simulink model "reachout_sample_spring"  (Simulink 8.1)
settings: Solver=ode4  SolverMode=SingleTasking  StartTime=0.0  StopTime=inf  FixedStep=0.0005  RelTol=1e-3
model workspace (MAT data in the model file):
  BKIN_STEP_TIME = 0.0005
  col_x = 1
  col_y = 2
  E_STAY_CENTER = 2
  E_TARGET_ON = 3
  E_HOLD_AT_TARGET = 5
  VRAD = 3
  LRAD = 4
  INIT_COLOR = 5
  REACH_COLOR = 6
  SHOULDER_VISC = 1
  ELBOW_VISC = 2
  START_TARGET = 1
  LOAD = 3
  DELAY_1ST_TARGET_FIXED = 4
  DELAY_1ST_TARGET_RANDOM = 5
  MAX_REACH_TIME = 6
  DELAY_2ND_TARGET = 7
  DELAY_POST_TRIAL = 8
  END_TARGET = 2
  A_VISC = 3
  B_VISC = 4
  C_VISC = 5
  D_VISC = 6
  X_SPRING = 7
  Y_SPRING = 8
  A_LINT = 9
  B_LINT = 10
  C_LINT = 11
  D_LINT : num (value not decoded)
StartFcn:
  |  warndlg('Dexterit-E models cannot run under simulation. Please compile your model and run it from within Dexterit-E.');set_param(bdroot,'SimulationCommand','stop')
libraries: General x3, KINARM_loads x3, Video x3, KINARM_general x2, KINARM_EP_loads x1
CloseFcn:
  | rtwprivate ssgencode ModelCloseRequest b2lab2d
settings Model: Creator=Chris Grebeldinger  LastModifiedBy=BKIN TECHNOLOGIES  ModifiedComment=chris -- Wed Feb 16 09:18:30 2005 -- Version 1.1384  ModifiedHistory=Feb 16/05 - Add error repeat, add offset ramp  ExtModeArmWhenConnect=off  ExtModeLogAll=off  BufferReuse=off
settings DataIOCC: LimitDataPoints=off  SaveOutput=off  SaveTime=off  SignalLoggingName=sigsOut
settings OptimizationCC: BlockReduction=off  BooleanDataType=off  OptimizeBlockIOStorage=off  BufferReuse=off  ExpressionFolding=off  FoldNonRolledExpr=off  LocalBlockOutputs=off  InitFltsAndDblsToZero=on
settings DebuggingCC: SaveWithParameterizedLinksMsg=none  SignalResolutionControl=TryResolveAllWithWarning  SolverPrmCheckMsg=none  MultiTaskDSMMsg=warning  MultiTaskCondExecSysMsg=none  StrictBusMsg=Warning
settings HardwareCC: ProdIntDivRoundTo=Zero  ProdEndianess=LittleEndian  ProdHWDeviceType=Generic->32-bit x86 compatible  TargetHWDeviceType=32-bit Generic
settings SFSimCC: SimCustomHeaderCode="#include \"stdlib.h\""  SFSimEcho=off  SimParseCustomCode=off
settings RTWCC: SystemTargetFile=xpctarget.tlc  TemplateMakefile=xpc_default_tmf  Description=xPC Target  ProcessScript=xpctarget_make_rtw_hook  CustomSourceCode="#include \"stdlib.h\""  IncludeERTFirstTime=on  RTWCompilerOptimization=On
settings CodeAppCC: MaxIdLength=63
settings xpcTargetCC: TargetFcnLib=ansi_tfl_tmw.mat  CodeReplacementLibrary=XPC_BLAS  ParMdlRefBuildCompliant=on  ConcurrentExecutionCompliant=on  CombineSignalStateStructs=off  MATLABClassNameForMDSCustomization=xpcAperiodicCustomization  GRTInterface=on  GenerateAllocFcn=off  xPCTaskExecutionProfile=off  xPCRL32EventNumber=5000  xPCisDownloadable=off  xPCisDefaultEnv=off  xPCLoadParamSetFile=off  xPCConcurrentTasks=off  xPCEnableSFAnimation=off

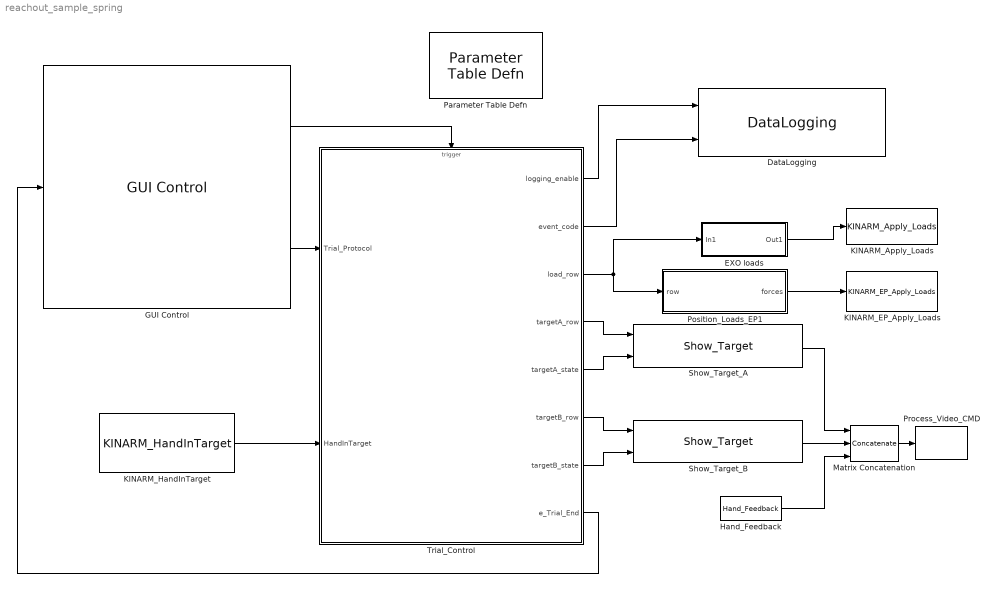
== system reachout_sample_spring ==
  DataLogging : General/DataLogging  log_event_codes=on  log_analog_inputs=off
      link override Poll KINARM/EPTorqueCMD: GotoTag=KINARMEPTorqueCMD
      link override Poll KINARM/TorqueCMD: GotoTag=KINARMTorqueCMD
  EXO loads : Subsystem
  GUI Control : General/GUI Control  target_type_str=Circle  Target_Type=1  XYcols=[1 2]  Vcols=3  Lcols=4  indices_padding=[0 0 0 0;0 0 0 0]  task_version=1.0  show_repeat_trial_flag=off
  Hand_Feedback : KINARM_general/Hand_Feedback  feedback_cntl_src=none
  KINARM_Apply_Loads : KINARM_loads/KINARM_Apply_Loads  up_duration=0  down_duration=0  max_torque=13
  KINARM_EP_Apply_Loads : KINARM_EP_loads/KINARM_EP_Apply_Loads  up_duration=1500  down_duration=1500  max_force=60
  KINARM_HandInTarget : KINARM_general/KINARM_HandInTarget  use_dominant_hand=on  target_type=Circle  num_states=1  attribcol1=[4]  attribcol2=[4]  attribcol3=[5]  attribcol4=[6]  attribcol5=[0]
  Matrix Concatenation : Concatenate  NumInputs=3  Mode=Multidimensional array
  Parameter Table Defn : General/Parameter Table Defn  ShowInLibBrowser=0
  Position_Loads_EP1 : Subsystem  AncestorBlock=KINARM_EP_loads/Velocity_Loads_EP  mask(Velocity_Loads_EP){use_dom_hand=on, loadcol=[A_VISC B_VISC C_VISC D_VISC X_SPRING Y_SPRING A_LINT B_LINT C_LINT D_LINT], source=dialog, scaling=1, stability=on}
      mask prompts: use_dom_hand "Load on dominant arm"; loadcol "Load Table columns [colA colB colC colD]"; source "Source for scaling"; stability "Suppress positive feedback"
      mask help:
      | <html><body>
      | The Velocity_Loads_EP block creates velocity dependent loads on the KINARM End-Point robot in a global cartesion coordinate frame, based on end-point (i.e. handle) velocity.
      |
      | <br><p>Hand force (N) is calculated as:
      | <br><p>Fx = A*Vx + B*Vy
      | <br>Fy = C*Vx + D*Vy
      | <br><p>where Vx and Vy are the x and y-direction fingertip velocities (m/s).
      |
      | <br><p>Parameters A,B,C,D in the above equations come from the Load Table, with the row determined by the "row" input to this block and the columns specified in the "Load Table columns" defined below.
      |
      | <br><p>The load can be scaled by a constant internal value or a Task Program-determined external value.  (Scaling of 1 = 100%)
      |
      | <br><p>Suppress positive feedback will ensure that A&lt;=0 and D&lt;=0 at run-time to avoid an unstable condition.
      |
      | <br><p><b>Warning</b> - Curl fields (valA=0, valB~=0, valC~=0, valD=0) should only be created with extreme care as they can lead to highly unstable situations.
      | </body></html>
      mask init:
      | library = 'KINARM_EP_loads';
      | numCol = 10;
      | [inputname1, inputname2, inputname3, outputname, columntext] = loadBlockInitCommands(gcb, library, numCol);
      mask Help:
      | Used to create a force vector for applying a velocity-dependent force field at the hand (fingertip).
      | 
      | <H2>Library </H2>
      | KINARM EP loads
      | 
      | <H2>Description </H2>
      | The Velocity_Loads_EP block creates velocity dependent loads on the KINARM End-Point robot in a global cartesion coordinate frame, based on end-point (i.e. handle) velocity.
      |  <P>
      | The force output of this block is filtered using a 50Hz 2nd-order Butterworth filter for stability.
      | <P>
      | The force field at the fingertip (N) is calculated as: <BR>
      | Fx = A*Vx + B*Vy <BR>
      | Fy = C*Vx + D*Vy <BR>
      | where Vx and Vy are the x and y-direction fingertip velocities (m/s).
      | <P>
      | For example, a viscous-based force field would be A=-0.5, B=0, C=0 D=-0.5.  The values of A, B, C and D are normally limited to between -20 and 20.  However, if secondary encoders are used, the values are limited to between -40 and 40.  Units of A, B, C and D are N/(m/s).
      | <br>For example, if the "row" input = 2, and "Load Table columns" are specifed as [1 2 3 4], then using the sample Load Table below, A = 1, B = 0.544, C = 2 and D = -1.
      | <br>
      | <tt>
      | __________________________________________<br>
      | |&nbsp;&nbsp;&nbsp;&nbsp;&nbsp;&nbsp;&nbsp;&nbsp;|Force A|Force B|Force C|Force D|<br>
      | ------------------------------------------<br>
      | | Load 1 |&nbsp;&nbsp;&nbsp;&nbsp;&nbsp;0 |&nbsp;&nbsp;&nbsp;&nbsp;&nbsp;0 |&nbsp;&nbsp;&nbsp;&nbsp;&nbsp;0 |&nbsp;&nbsp;&nbsp;&nbsp;&nbsp;0 |<br>
      | | Load 2 |&nbsp;&nbsp;&nbsp;&nbsp;&nbsp;1 | 0.544 |&nbsp;&nbsp;&nbsp;&nbsp;&nbsp;2 |&nbsp;&nbsp;&nbsp;&nbsp;-1 |<br>
      | | Load 3 |&nbsp;&nbsp;&nbsp;&nbsp;-2 |&nbsp;&nbsp;&nbsp;&nbsp;&nbsp;0 |&nbsp;&nbsp;&nbsp;&nbsp;-2 |&nbsp;&nbsp;&nbsp;&nbsp;&nbsp;0 |<br>
      | ------------------------------------------<br>
      | </tt>
      | <P>
      | <B>row: </B> this scalar input indicates which row in the Load Table the coefficients [A, B, C, D] will come from.
      | <P>
      | <B>Scaling: </B> this scalar input is only present if 'port' source for scaling has been chosen in the dialog box (see below).  When it is present, the actual value of the loads output from this block are scaled by this input.  For 100% of desired load, scaling=1.
      | <P>
      | <B>Forces: </B> this vector output is in global, cartesian coordinate space.  It must be wired to the KINARM_EP_Apply_Loads block to actually apply the loads to the KINARM End-Point.  This output may be added to other Force outputs from other KINARM End-Point load blocks to create a composite load.
      | <P>
      | 
      | 
      | 
      | <H2>Parameters and Dialog Box</H2>
      | <P>
      | <B>Load on Dominant Arm:</B> indicates whether or not this load is applied to the dominant arm (checked box) or non-dominant arm (unchecked box). .
      | <P>
      | <B>Load Table Columns: </B> needs to be a 4x1 vector with the vector elements corresponding to the columns in the Load Table for parameters A, B, C and D.  If a parameter is not going to be in the Load Table, then the value 0 should be used in the "Load Table Columns" vector  (e.g. if only viscous loads are specified in the Load Table, and the viscous parameter are in columns 2 and 3, then the "Load Table Columns" vector should be [2 0 0 3], which indicates that B and C are not specified in the Load Table and so both B and C are set =0).
      | <P>
      | <B>Source for scaling: </B> refers to the source for scaling of the load.  If the source is dialog, then a Scaling option appears in the Dialog box.  If the source is port, then a new input appears to this Simulink block.  For loads that are always on, use a dialog scale with the value set to 1.  For loads that need to be controlled by the Task Program machine (e.g. to turn them on or off) or by an external block (e.g. to ramp up a load), use a port source for the scaling.
      | <P>
      | <B>Scaling: </B>  this dialog input is only present if 'dialog' source for scaling has been chosen in the dialog box.  When it is present, the actual value of the loads output from this block are scaled by this input.  For 100% of desired load, scaling=1.
      | <P>
      | <B>Suppress Positive Feedback: </B> if checked will suppress potentially unstable loads at runtime.  These include forcing A&lt;=0 and D&lt;=0 (i.e. only allow resistive viscosity coefficients).
      | <P>
      | 
      | <H2>Related Blocks </H2>
      | KINARM_EP_Apply_Loads<BR>
      | Velocity_loads_EP_(inter-arm)<BR>
      mask Callback loadcol:
      | %%%%
      | % Because of bugs iN R2007, R2010a and R2013a (which have been reported to Mathworks), the following code
      | % is required here because in the Initialization Section it will ONLY correctly update those Mask Parameters that are hidden
      | % when the OK button is clicked (NOTE: the initialization code will correctly update all Mask Parameters when the Apply button
      | % is clicked, the bug is that it should also update everything when the OK button is clicked in the absence of an Apply click)
      | %
      | % Adding a set_param call which updates one of the mask parameters will call the initialization code to run, which "avoids"
      | % this bug. This code should be removed once Mathworks has fixed this bug.
      | 
      | temp = get_param(gcb, 'loadcol');
      | set_param(gcb, 'loadcol', temp);
      mask TypeOptions source: dialog | port
      mask Callback source:
      | sourceStr=get_param(gcb,'source');
      | vis=get_param(gcb,'MaskVisibilities');
      | 
      | if strmatch(sourceStr, 'dialog')
      | 	vis{4}='on';
      | else
      | 	vis{4}='off';
      | end
      | 
      | set_param(gcb,'MaskVisibilities',vis);
      mask Display: disp(columntext); port_label('output',1,outputname); port_label('input',1, inputname1);
  Process_Video_CMD : Video/Process_Video_CMD
  Show_Target_A : Video/Show_Target  target_type=Circle  num_states=2  attribcol1=[INIT_COLOR 0 0 VRAD]  attribcol2=[REACH_COLOR 0 0 VRAD]  attribcol3=[0 0 0 0]  attribcol4=[0 0 0 0]  attribcol5=[0 0 24 0]  stateindices_padding=[0 0 0 0 0 0 0;0 0 0 0 0 0 0;0 0 0 0 0 0 0;0 0 0 0 0 0 0;0 0 0 0 0 0 0]  source=dialog  opacity=100  target_display=Both subject and operator displays  num_col=4
  Show_Target_B : Video/Show_Target  target_type=Circle  num_states=2  attribcol1=[INIT_COLOR 0 0 VRAD]  attribcol2=[REACH_COLOR 0 0 VRAD]  attribcol3=[0 0 0 0]  attribcol4=[0 0 0 0]  attribcol5=[0 0 24 0]  stateindices_padding=[0 0 0 0 0 0 0;0 0 0 0 0 0 0;0 0 0 0 0 0 0;0 0 0 0 0 0 0;0 0 0 0 0 0 0]  source=dialog  opacity=100  target_display=Both subject and operator displays  num_col=4
  Trial_Control : Stateflow chart  TreatAsAtomicUnit=on
  wires:
  KINARM_HandInTarget/1 -> Trial_Control/2(HandInTarget)
  Show_Target_A/1 -> Matrix Concatenation/1
  GUI Control/2 -> Trial_Control/1(Trial_Protocol)
  Trial_Control/8(e_Trial_End) -> GUI Control/1
  GUI Control/1 -> Trial_Control/Trigger
  Trial_Control/5(targetA_state) -> Show_Target_A/2
  Trial_Control/4(targetA_row) -> Show_Target_A/1
  Matrix Concatenation/1 -> Process_Video_CMD/1
  Hand_Feedback/1 -> Matrix Concatenation/3
  Show_Target_B/1 -> Matrix Concatenation/2
  Trial_Control/6(targetB_row) -> Show_Target_B/1
  Trial_Control/7(targetB_state) -> Show_Target_B/2
  Trial_Control/3(load_row) -> Position_Loads_EP1/1(row), EXO loads/1(In1)
  Trial_Control/1(logging_enable) -> DataLogging/1
  Trial_Control/2(event_code) -> DataLogging/2
  EXO loads/1(Out1) -> KINARM_Apply_Loads/1
  Position_Loads_EP1/1(forces) -> KINARM_EP_Apply_Loads/1

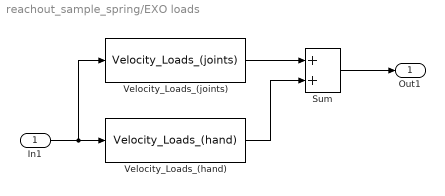
== system reachout_sample_spring/EXO loads ==
  In1 : Inport
  Sum : Sum
  Velocity_Loads_(hand) : KINARM_loads/Velocity_Loads_(hand)  use_dom_hand=on  loadcol=[A_VISC B_VISC C_VISC D_VISC]  source=dialog  scaling=1  stability=on
  Velocity_Loads_(joints) : KINARM_loads/Velocity_Loads_(joints)  use_dom_hand=on  loadcol=[SHOULDER_VISC 0 0 ELBOW_VISC]  source=dialog  scaling=1  stability=on
  Out1 : Outport
  wires:
  In1/1 -> Velocity_Loads_(joints)/1, Velocity_Loads_(hand)/1
  Sum/1 -> Out1/1
  Velocity_Loads_(joints)/1 -> Sum/1
  Velocity_Loads_(hand)/1 -> Sum/2

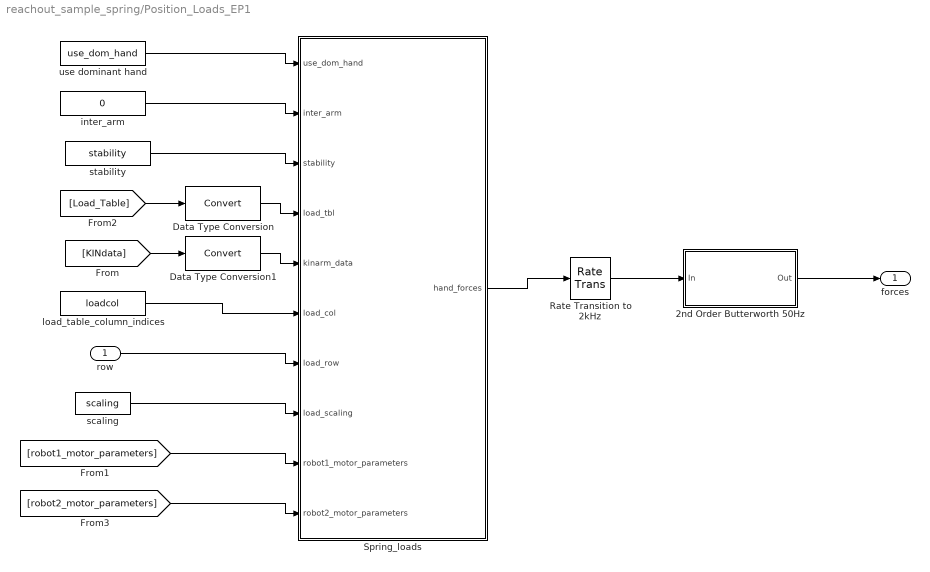
== system reachout_sample_spring/Position_Loads_EP1 ==
  row : Inport
  2nd Order Butterworth 50Hz : Subsystem
  Data Type Conversion : DataTypeConversion
  Data Type Conversion1 : DataTypeConversion
  Rate Transition to 2kHz : RateTransition  OutPortSampleTime=.0005
  Spring_loads : MATLAB Function  TreatAsAtomicUnit=on
  inter_arm : Constant  Value=0
  load_table_column_indices : Constant  Value=loadcol
  scaling : Constant  Value=scaling
  stability : Constant  Value=stability
  use dominant hand : Constant  Value=use_dom_hand
  forces : Outport
  wires:
  Data Type Conversion1/1 -> Spring_loads/5(kinarm_data)
  Data Type Conversion/1 -> Spring_loads/4(load_tbl)
  Rate Transition to 2kHz/1 -> 2nd Order Butterworth 50Hz/1(In)
  [robot2_motor_parameters] -> Spring_loads/10(robot2_motor_parameters)
  [robot1_motor_parameters] -> Spring_loads/9(robot1_motor_parameters)
  2nd Order Butterworth 50Hz/1(Out) -> forces/1
  use dominant hand/1 -> Spring_loads/1(use_dom_hand)
  [Load_Table] -> Data Type Conversion/1
  [KINdata] -> Data Type Conversion1/1
  row/1 -> Spring_loads/7(load_row)
  load_table_column_indices/1 -> Spring_loads/6(load_col)
  Spring_loads/1(hand_forces) -> Rate Transition to 2kHz/1
  stability/1 -> Spring_loads/3(stability)
  inter_arm/1 -> Spring_loads/2(inter_arm)
  scaling/1 -> Spring_loads/8(load_scaling)

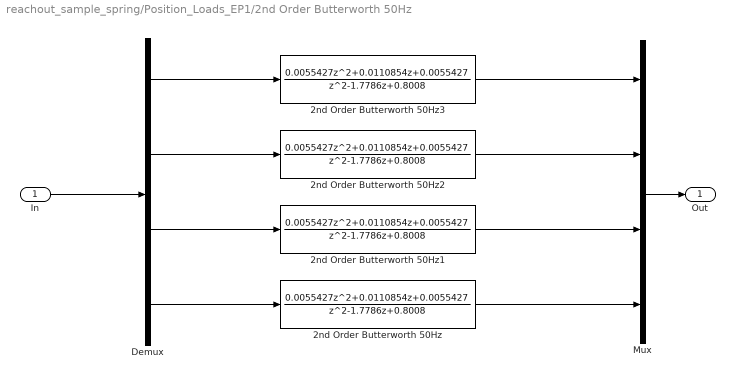
== system reachout_sample_spring/Position_Loads_EP1/2nd Order Butterworth 50Hz ==
  In : Inport
  2nd Order Butterworth 50Hz{,1..3} (4 alike) : DiscreteTransferFcn  Numerator=[0.0055427 0.0110854 0.0055427]  Denominator=[1 -1.7786 0.8008]
  Demux : Demux
  Mux : Mux
  Out : Outport
  wires:
  Demux/1 -> 2nd Order Butterworth 50Hz3/1
  Demux/2 -> 2nd Order Butterworth 50Hz2/1
  Demux/3 -> 2nd Order Butterworth 50Hz1/1
  Demux/4 -> 2nd Order Butterworth 50Hz/1
  In/1 -> Demux/1
  Mux/1 -> Out/1
  2nd Order Butterworth 50Hz3/1 -> Mux/1
  2nd Order Butterworth 50Hz2/1 -> Mux/2
  2nd Order Butterworth 50Hz1/1 -> Mux/3
  2nd Order Butterworth 50Hz/1 -> Mux/4

== stateflow chart Trial_Control ==
  settings: sampleTime=0.001
  state Inter_Trial_State/
    // Turn off both targets, turn off data logging, reset the
    // event code, and send the e_Trial_End Stateflow event.
    event_code = 0;
    targetA_state = 0;
    targetB_state = 0;
    logging_enable = 0;
    e_Trial_End;
  state Initialize/
    // Both the targets and data logging are initially off.
    targetA_state = 0;
    targetB_state = 0;
    logging_enable = 0;
  state MainTrial
    state ShowSecondTarget/
      // Turn on second target and log an event indicating this has occurred. Then wait until the hand is the target or until a specified time has elapsed.
      event_code = E_TARGET_ON;
      targetB_row = Trial_Protocol[END_TARGET];
      targetB_state = 1;
      tickCount = Trial_Protocol[MAX_REACH_TIME];
    state StayAtSecondTarget/
      // Log an event that the second target was reached, change that target's state, and then wait for a specified time.
      event_code = E_HOLD_AT_TARGET;
      targetB_state = 2;
      tickCount = Trial_Protocol[DELAY_2ND_TARGET];
    state EndOfTrial/
      // Set the post-trial delay.
      tickCount = Trial_Protocol[DELAY_POST_TRIAL];
    state StayAtFirstTarget/
      // Log an event that target was reached, begin data logging, change the first target's state, and then wait for a specified time.
      // The wait time may have both a fixed and a random component. The hand must stay in the target for the full wait time.
      logging_enable = 1;
      event_code = E_STAY_CENTER;
      targetA_state = 2;
      tickCount = Trial_Protocol[DELAY_1ST_TARGET_FIXED] + Trial_Protocol[DELAY_1ST_TARGET_RANDOM] * rand() / RAND_MAX;
    state ShowFirstTarget/
      // Turn on first target, set loading conditions, enable data logging, and wait for a specified time or until the hand is in the target.
      targetA_row = Trial_Protocol[START_TARGET];
      targetA_state = 1;
      load_row = Trial_Protocol[LOAD];
    ShowFirstTarget -> StayAtFirstTarget : [HandInTarget[targetA_row] == 1]
    StayAtFirstTarget -> ShowFirstTarget [order 2] : [HandInTarget[targetA_row] == 0]
    StayAtFirstTarget -> ShowSecondTarget [order 1] : after(tickCount, e_clk)
    ShowSecondTarget -> StayAtSecondTarget [order 2] : [HandInTarget[targetB_row]==1]
    ShowSecondTarget -> EndOfTrial [order 1] : after(tickCount, e_clk)
    StayAtSecondTarget -> EndOfTrial : after(tickCount, e_clk)
  (default) -> Initialize
  Initialize -> ShowFirstTarget
  Inter_Trial_State -> ShowFirstTarget : after(tickCount, e_clk)
  MainTrial -> Inter_Trial_State : e_ExitTrialNow/
      | tickCount = 1;
  EndOfTrial -> Inter_Trial_State
  data: logging_enable output boolean; Trial_Protocol input double; HandInTarget input double; event_code output uint16 [0..] =0; load_row output double [1..32]; targetA_row output double [1..32]; targetA_state output double; targetB_row output double; targetB_state output double; tickCount local double; RAND_MAX constant double =32767
  data load_row settings: description=current index into the loadtable
  data targetA_row settings: description=index of the row currently being used in the TargetTable
  events: e_clk input RISING_EDGE_EVENT; e_ExitTrialNow input EITHER_EDGE_EVENT; e_Trial_End output EITHER_EDGE_EVENT

== matlab function Position_Loads_EP1/Spring_loads ==
  data: use_dom_hand input double; hand_forces output double; inter_arm input double; stability input double; load_tbl input double; kinarm_data input double; load_col input double; load_row input double; load_scaling input double; robot1_motor_parameters input double; robot2_motor_parameters input double
function hand_forces  = hand_pos_loads(use_dom_hand, inter_arm, stability, load_tbl, kinarm_data, load_col, load_row, load_scaling, robot1_motor_parameters, robot2_motor_parameters)
%
% HAND-SPACE VELOCITY DEPENDENT FORCE FIELD 
%
% revision 3
%


% Maximum velocity feedback gains
max_gain_secondary = 40;   %for secondary encoders
max_gain_primary = 20;     %for primary encoders



% kinarm_data indicies
L1_index = 1;				% L1
L2_index = 2;				% L2
L2ptr_index=3;				% L2 pointer (finger tip offset)
ORIENT_index = 6;			% 1=right	2=left
SHOANG_index = 7;			% Shoulder angle
ELBANG_index = 8;			% Elbow angle
HXPOS_index = 23;			% Hand x position
HYPOS_index = 24;			% Hand y position
SHOVEL_FILT_index = 35;		% filtered velocities
ELBVEL_FILT_index = 36;



% by default, all loads are zeroed
hand_forces = [0,0,0,0];


%determine which arm to apply the load to
dominant_hand=kinarm_data(3,1);						%kinarm_data(3,1) tells which arm is the dominant arm
if use_dom_hand==1
	loading_arm=dominant_hand;
else
	loading_arm=3-dominant_hand;
end

%if inter_arm==0, then loading and feedback occur on same arm.  
%if inter_arm==1, then feedback comes from other arm (i.e. loading occurs
%on hand specified in Mask)
if inter_arm==0
    feedback_arm=loading_arm
else
    feedback_arm=3-loading_arm
end

% check to see which type of encoder is present on the feedback arm
% if the feedback arm is arm 1, then set the secondary encoder flag for robot 1
% if the feedback arm is arm 2, then set the secondary encoder flag for robot 2
% if sec_enc_feedbackarm==0, then primary encoders are used on the feedback arm
% if sec_enc_feedbackarm==1, then secondary encoders are used on the feedback arm
if feedback_arm==1
    sec_enc_feedbackarm = robot1_motor_parameters(6);
else
    sec_enc_feedbackarm = robot2_motor_parameters(6);
end


if load_row > 0 && load_row <= size(load_tbl,1)
	CA=0;	CB=0;	CC=0;	CD=0;		%default values
	% global frame force field coefficients    
	if load_col(1)>0
		CA = load_tbl( load_row, load_col(1));
	end
	if load_col(2)>0
		CB = load_tbl( load_row, load_col(2));
	end
	if load_col(3)>0
		CC = load_tbl( load_row, load_col(3));
	end
	if load_col(4)>0
		CD = load_tbl( load_row, load_col(4));
	end
	if stability==1		%force stability for viscous loads
		CA=min(CA,0);
		CD=min(CD,0);
    end
    
    xk_center = load_tbl( load_row,load_col(5));
    yk_center = load_tbl( load_row,load_col(6));

    % limit the velocity feedback gains
    % if the feedback arm has secondary encoders, then limit the gain to the maximum secondary encoder gain
    % if the feedback arm has primary encoders, then limit the gain to the maximum primary encoder gain   
    if sec_enc_feedbackarm == 1
        if CA<-max_gain_secondary
            CA=-max_gain_secondary
        end
        if CB<-max_gain_secondary
            CB=-max_gain_secondary
        end
        if CC<-max_gain_secondary
            CC=-max_gain_secondary
        end
        if CD<-max_gain_secondary
            CD=-max_gain_secondary
        end
        if CA>max_gain_secondary
            CA=max_gain_secondary
        end
        if CB>max_gain_secondary
            CB=max_gain_secondary
        end
        if CC>max_gain_secondary
            CC=max_gain_secondary
        end
        if CD>max_gain_secondary
            CD=max_gain_secondary
        end
    else
        if CA<-max_gain_primary
            CA=-max_gain_primary
        end
        if CB<-max_gain_primary
            CB=-max_gain_primary
        end
        if CC<-max_gain_primary
            CC=-max_gain_primary
        end
        if CD<-max_gain_primary
            CD=-max_gain_primary
        end
        if CA>max_gain_primary
            CA=max_gain_primary
        end
        if CB>max_gain_primary
            CB=max_gain_primary
        end
        if CC>max_gain_primary
            CC=max_gain_primary
        end
        if CD>max_gain_primary
            CD=max_gain_primary
        end
    end
        

    % Build rotation matrix
    R_mat = [load_tbl( load_row,load_col(7)) load_tbl( load_row,load_col(8));
             load_tbl( load_row,load_col(9)) load_tbl( load_row,load_col(10))];
    
    
	%---------------------------------------------------------------
	% define the x and y velocities
	HXPOS = kinarm_data( feedback_arm, HXPOS_index );
	HYPOS = kinarm_data( feedback_arm, HYPOS_index );

	%-----------------------------------------------------------------
	% calculate force field force components
    hf = [CA*(HXPOS + xk_center) + CB*(HYPOS + yk_center);
          CC*(HXPOS + xk_center) + CD*(HYPOS + yk_center)];
    hf = R_mat * hf;
    
    hand_forces(1+2*(loading_arm-1)) = hf(1);
    hand_forces(2+2*(loading_arm-1)) = hf(2);
    
% 	hand_forces(1+2*(loading_arm-1))=CA*(HXPOS + xk_center) + CB*(HYPOS + yk_center);			%FX
% 	hand_forces(2+2*(loading_arm-1))=CC*(HXPOS + xk_center) + CD*(HYPOS + yk_center);			%FY
    


end
hand_forces=hand_forces*load_scaling;
